simulink model "SLX_Read"  (R2026a)
settings: Solver=VariableStepAuto
values from neighbouring files (symbols this model uses):
  g = 9.81    [paramsForTask2.m]
  J = 1    [paramsForTask2.m]
  m = 200    [paramsForTask2.m]
  R = 0.3    [paramsForTask2.m]
  v0 = 25    [paramsForTask2.m]
settings Model: SILPILModeSetting=veronly  Creator=Josh  LastModifiedBy=Josh
settings RTWCC: BuildConfiguration=Faster Runs

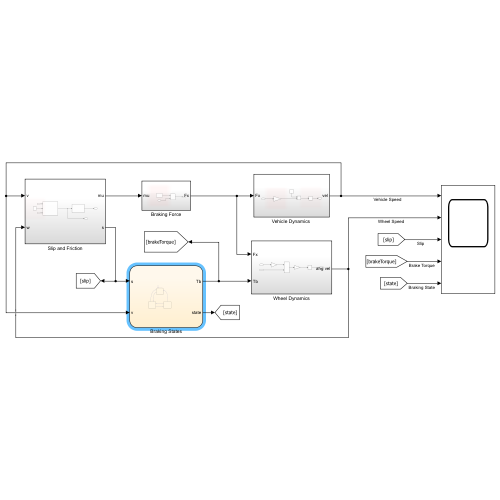
[thumbnail: Simulink's stored preview of the top-level diagram]
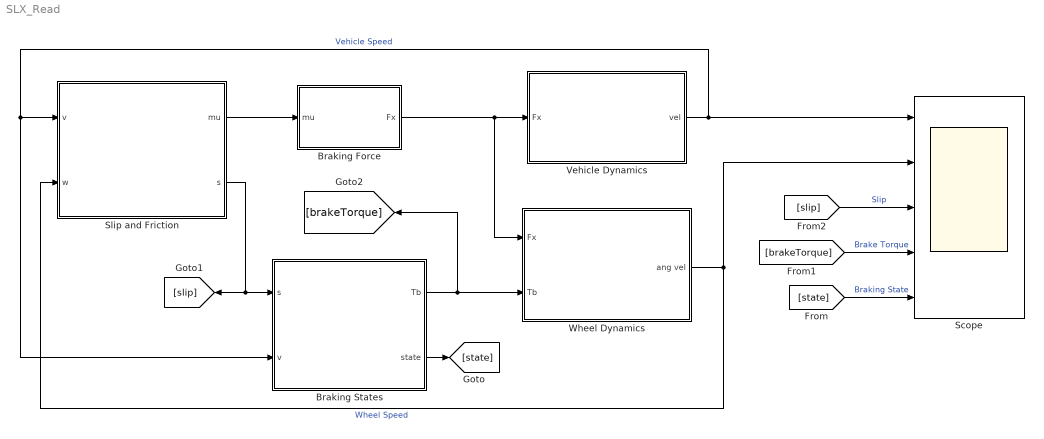
== system SLX_Read ==
  Braking Force : Subsystem
  Braking States : Stateflow chart  TreatAsAtomicUnit=on
  Scope : Scope  NumInputPorts=5
      settings: ActiveDisplayYMinimum=-2.1898282670968321  ActiveDisplayYMaximum=40.5141729181734
  Slip and Friction : Subsystem
  "Vehicle Dynamics " : Subsystem
  Wheel Dynamics : Subsystem
  wires:
  Braking States/1(Tb) -> Wheel Dynamics/2(Tb), [brakeTorque]
  "Vehicle Dynamics "/1(vel) -> Slip and Friction/1(v), Braking States/2(v), Scope/1  "Vehicle Speed"
  Slip and Friction/1(mu) -> Braking Force/1(mu)
  Braking Force/1(Fx) -> "Vehicle Dynamics "/1(Fx), Wheel Dynamics/1(Fx)
  Slip and Friction/2(s) -> Braking States/1(s), [slip]
  Braking States/2(state) -> [state]
  [state] -> Scope/5  "Braking State"
  [slip] -> Scope/3  "Slip"
  [brakeTorque] -> Scope/4  "Brake Torque"
  Wheel Dynamics/1(ang vel) -> Scope/2, Slip and Friction/2(w)  "Wheel Speed"

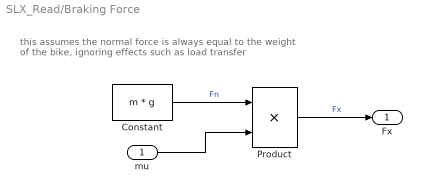
== system SLX_Read/Braking Force ==
  note: this assumes the normal force is always equal to the weight of the bike, ignoring effects such as load transfer
  mu : Inport
  Constant : Constant  Value=m * g
  Product : Product
  Fx : Outport
  wires:
  Constant/1 -> Product/1  "Fn"
  mu/1 -> Product/2
  Product/1 -> Fx/1  "Fx"

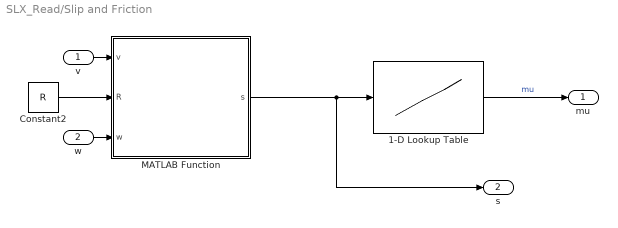
== system SLX_Read/Slip and Friction ==
  v : Inport
  w : Inport  Port=2
  1-D Lookup Table : Lookup_n-D  NumberOfTableDimensions=1  BreakpointsForDimension1=[0;5;10;15;20;30;50;100] ./ 100  Table=[0;0.59999999999999998;0.90000000000000002;1;0.94999999999999996;0.75;0.40000000000000002;0.10000000000000001]  InternalRulePriority=Speed  RndMeth=Simplest
  Constant2 : Constant  Value=R
  MATLAB Function : MATLAB Function  TreatAsAtomicUnit=on
  mu : Outport
  s : Outport  Port=2
  wires:
  MATLAB Function/1(s) -> s/1, 1-D Lookup Table/1
  Constant2/1 -> MATLAB Function/2(R)
  v/1 -> MATLAB Function/1(v)
  1-D Lookup Table/1 -> mu/1  "mu"
  w/1 -> MATLAB Function/3(w)

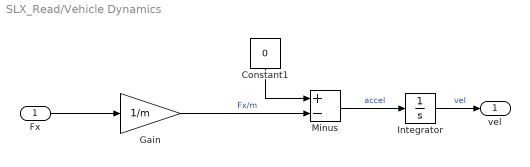
== system SLX_Read/Vehicle Dynamics  ==
  Fx : Inport
  Constant1 : Constant  Value=0
  Gain : Gain  Gain=1/m
  Integrator : Integrator  InitialCondition=v0
  Minus : Sum  Inputs=+-
  vel : Outport
  wires:
  Integrator/1 -> vel/1  "vel"
  Minus/1 -> Integrator/1  "accel"
  Gain/1 -> Minus/2  "Fx/m"
  Constant1/1 -> Minus/1
  Fx/1 -> Gain/1

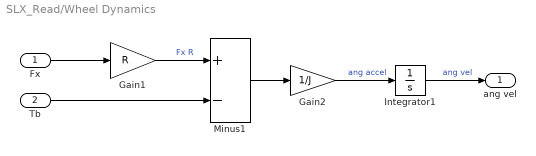
== system SLX_Read/Wheel Dynamics ==
  Fx : Inport
  Tb : Inport  Port=2
  Gain1 : Gain  Gain=R
  Gain2 : Gain  Gain=1/J
  Integrator1 : Integrator  InitialCondition=v0/R
  Minus1 : Sum  Inputs=+-
  ang vel : Outport
  wires:
  Tb/1 -> Minus1/2
  Minus1/1 -> Gain2/1
  Integrator1/1 -> ang vel/1  "ang vel"
  Gain1/1 -> Minus1/1  "Fx R"
  Gain2/1 -> Integrator1/1  "ang accel"
  Fx/1 -> Gain1/1

== matlab function SLX_Read/Slip and Friction/MATLAB Function ==
  data: v input; R input; s output; w input
function s = calcSlip(v, R, w)
    s = (v - w*R) / v;  % this is ok if v is never 0
end

== stateflow chart SLX_Read/Braking States ==
  note: please note you will have to install stateflow to run this part of the simulation if you do not have it already. sorry for inconvenience
  state INACTIVE
    entry:
    Tb = 0;
    state = 0;
  state BRAKING
    entry:
    Tb = 700;
    state = 1;
  state ABS_ACTIVE
    entry:
    Tb = 400;
    state = 2;
  note: here i have assumed the braking torque values as they were not given. with abs active braking torque is reduced by 400Nm
  (default) -> state1
  state3 -> state1 [order 2] : [v <= 10]
  state4 -> state1 [order 2] : [v <= 10]
  state1 -> state3 : [v > 10]
  state4 -> state3 [order 1] : [s < 0.10]
  state3 -> state4 [order 1] : [s > 0.15]
  data: s input double; Tb output double; state output double; v input double
